simulink model "mu_nonlinear_sim"  (R2026b)
settings: Solver=VariableStepAuto
InitFcn:
  | seaDir=fileparts(get_param(bdroot,'FileName'));if isfile(fullfile(seaDir,'..','collaudo_simulink.m')),addpath(fullfile(seaDir,'..'));else,addpath(fullfile(seaDir,'..','..','File_di_Funzioni_Progetto-Accorpati'));end;collaudo_simulink(bdroot);
model workspace (MAT data in the model file):
  A = [0  0  1  0  0  0  0  0  0  0  0  0  0  0; 0  0  0  1  0  0  0  0  0  0  0  0  0  0; -287.975  563.713333333  0  0  312.5  -583.333333333  0  0  0  0  0  0  0  0; 704.641666667  -1838.18666667  0  0  -729.166666667  1916.66666667  0  0  0  0  0  0  0  0; 0  0  0  0  0  0  1  0  0  0  0  0  0  0; 0  0  0  0  0  0  0  1  0  0  0  0  0  0; 5000  0  0  0  -5000  0  -2  0  0  -156.25  651.041666667  0  0  0; 0  4000  0  0  0  -4000  0  -2  0  0  0  0  -156.25  651.041666667; 0  0  0  0  0  0  0  0  -197.333333333  -79.1666666667  -52.0833333333  0  0  0; 0  0  0  0  0  0  0  0  128  0  0  0  0  0; 0  0  0  0  0  0  0  0  0  32  0  0  0  0; 0  0  0  0  0  0  0  0  0  0  0  -197.333333333  -79.1666666667  -52.0833333333; 0  0  0  0  0  0  0  0  0  0  0  128  0  0; 0  0  0  0  0  0  0  0  0  0  0  0  32  0]
  Ak1 = [-59053.7551233 -15060.4417981 -247384.802166 -33683.9989112 -58744.8100055 -15054.8155194 -240737.427005 -34798.0678804 -380.093427931 -2.64528507321e-11 -2.86785014033e-11 -70.1772916652 ... (324 elements, 18x18)]
  Ak2 = [-66482.5138518 58859.9072435 -3939180219.02 8861329774.8 0.00962184169638 0.0021126060022 -0.307210144554 -0.149393411391 -808382.886676 -1.97154781154e-06 -5.5678995061e-07 -402416.605778 ... (484 elements, 22x22)]
  Aplant = [0  0  1  0  0  0  0  0  0  0  0  0  0  0; 0  0  0  1  0  0  0  0  0  0  0  0  0  0; -287.975  563.713333333  0  0  312.5  -583.333333333  0  0  0  0  0  0  0  0; 704.641666667  -1838.18666667  0  0  -729.166666667  1916.66666667  0  0  0  0  0  0  0  0; 0  0  0  0  0  0  1  0  0  0  0  0  0  0; 0  0  0  0  0  0  0  1  0  0  0  0  0  0; 5000  0  0  0  -5000  0  -2  0  0  -156.25  651.041666667  0  0  0; 0  4000  0  0  0  -4000  0  -2  0  0  0  0  -156.25  651.041666667; 0  0  0  0  0  0  0  0  -197.333333333  -79.1666666667  -52.0833333333  0  0  0; 0  0  0  0  0  0  0  0  128  0  0  0  0  0; 0  0  0  0  0  0  0  0  0  32  0  0  0  0; 0  0  0  0  0  0  0  0  0  0  0  -197.333333333  -79.1666666667  -52.0833333333; 0  0  0  0  0  0  0  0  0  0  0  128  0  0; 0  0  0  0  0  0  0  0  0  0  0  0  32  0]
  B = [0  0; 0  0; 0  0; 0  0; 0  0; 0  0; 0  0; 0  0; 8  0; 0  0; 0  0; 0  8; 0  0; 0  0]
  Bk1 = [-41971.7925923  -11081.1547486; -10702.5482864  -2862.34383586; -175622.627059  -46334.0254179; -24431.1418067  -6701.2370812; -41752.2098485  -11023.2672925; -10698.572028  -2860.7387349; -174656.417143  -46079.7084794; -24722.2969121  -6774.18550393; 2.40651657511e-11  6.37680376741e-12; -1.88006601576e-11  -4.97364228434e-12; -2.03813396558e-11  -5.41993380938e-12; 1.08535358931e-11  2.8764122053e-12; 9.45959622107e-14  1.502238924e-14; 6.09740887216e-12  1.59629499127e-12; 1  4.38779674844e-13; -1.60225617681e-11  0.999999999996; 2.09437869826e-11  5.51387120759e-12; 7.22259613326e-12  1.92024020066e-12]
  Bk2 = [-1.469715923e-05  -5.03392161697e-06  66481.5344792  -58860.9820595; -1.60967680897e-05  -5.61949285195e-06  -58860.9820595  240347.325722; 0.0248933110796  0.0149679212434  3939075365.52  -9206373341.64; -2.94053204371  -1.03244143942  -8861110672.09  30611501156.9; 8.38580299227e-11  2.88681171192e-11  -0.00961625066757  -0.0107019560654; 1.81369365811e-11  6.22825118722e-12  -0.00211139708193  -0.00220551516129; -2.44265911788e-09  -8.38310293341e-10  5000.30704734  0.311108840593; -1.28586131714e-09  -4.47766304456e-10  0.149307574964  4000.17933035; -3.3652681538e-15  -7.79427381522e-16  1.22929631189e-07  5.43969913477e-07; -1.54732535343e-14  -5.27443674215e-15  1.97051724139e-06  1.69233324755e-06; -5.91421615725e-15  -1.60957708692e-15  5.56404379394e-07  6.44318326468e-07; 6.60057972656e-15  2.06268116455e-15  -1.4300097113e-07  -1.54855124633e-06; -2.97654953502e-15  2.4134857998e-16  -3.49285009668e-07  4.31276255736e-07; -2.94350008791e-14  -1.06328803069e-14  3.2069323084e-06  4.47049231709e-06; 2  -2.928912043e-15  9.46335392933e-07  1.16503477027e-06; 2.28965391755e-14  7.37138472727e-15  -2.63923776257e-06  -2.83353275499e-06; 4.99201069125e-16  2  -6.74353253191e-08  -1.3033050226e-07; 2.3272465043e-15  7.76116322822e-16  -2.74324508576e-07  -3.61337801409e-07; -1.06347642829e-12  -3.65803490785e-13  1.00012374907  0.000134433844037; -3.40933375091e-13  -1.18005737123e-13  3.9069788798e-05  1.00004517384; 3.33367848603e-15  1.22297283889e-15  -4.2121398571e-07  -3.40032598636e-07; 2.80802881661e-16  3.33510230464e-16  -8.09517197876e-08  -4.97664970119e-08]
  Bplant = [0  0  0  0  0  0  0  0; 0  0  0  0  0  0  0  0; 0  0  6.25  -14.5833333333  6.25  -14.5833333333  0  0; 0  0  -14.5833333333  47.9166666667  -14.5833333333  47.9166666667  0  0; 0  0  0  0  0  0  0  0; 0  0  0  0  0  0  0  0; 0  0  0  0  0  0  0  0; 0  0  0  0  0  0  0  0; 8  0  0  0  0  0  8  0; 0  0  0  0  0  0  0  0; 0  0  0  0  0  0  0  0; 0  8  0  0  0  0  0  8; 0  0  0  0  0  0  0  0; 0  0  0  0  0  0  0  0]
  C = [1  0  0  0  0  0  0  0  0  0  0  0  0  0; 0  1  0  0  0  0  0  0  0  0  0  0  0  0; 0  0  0  0  1  0  0  0  0  0  0  0  0  0; 0  0  0  0  0  1  0  0  0  0  0  0  0  0]
  Ck1 = [-47.5116784914  -5.78209213287  -5.13823657239  -1.08700411022  -2.20352010323  2.66425180559  -0.125034922339  0.185992241592  -0.927741743434  -1.56246668763  -3.63799575165  0.692641920355  1.31947037114  4.18733038989  131.03488926  -0.481581356595  185.834513399  7.27974776868; -8.77216145816  -28.2907119683  -1.33504865248  -1.92106436843  2.82254774196  -9.29393606241  0.15386065621  -0.640740236363  0.661174214458  1.22612259058  3.63119486569  -2.61713226851  -4.77953727904  -14.316530373  8.32978038536  120.88787202  7.40561859226  167.361916298]
  Ck2 = [-101047.860834  -35271.4725267  -10213.2861669  -3422.70914383  -726.305194157  -2764.75614997  -134.44732536  -147.179762398  -1026.38324203  -1695.61454007  -3888.56222989  -577.341883828  -1018.80852496  -3004.81089551  37664.9906718  104577.837385  12946.0064238  38967.5403937  -276393.79928  -109642.430073  -16958.192986  -8226.89474918; -50302.0757223  -17755.3765506  -5087.46688004  -1714.88123493  -339.218722956  -1461.38985543  -65.6273114827  -77.9347122137  -507.469938959  -837.275262695  -1911.06705358  -299.403482778  -530.388353735  -1580.54605831  18756.946896  52040.0304562  6501.42413314  19681.1036111  -137452.475336  -55605.1885505  -8506.38250139  -4027.49208907]
  Cplant = [1  0  0  0  0  0  0  0  0  0  0  0  0  0; 0  1  0  0  0  0  0  0  0  0  0  0  0  0; 0  0  0  0  1  0  0  0  0  0  0  0  0  0; 0  0  0  0  0  1  0  0  0  0  0  0  0  0]
  D = [0  0; 0  0; 0  0; 0  0]
  Dk1 = [0  0; 0  0]
  Dk2 = [0  0  0  0; 0  0  0  0]
  Dplant = [0  0  0  0  0  0  0  0; 0  0  0  0  0  0  0  0; 0  0  0  0  0  0  0  0; 0  0  0  0  0  0  0  0]
  Gact = ss
  Gact.IOSize_ = [1 1]
  Gact.Data_ = ltipack.ssdata
  Gact.Data_.a = [-197.333333333  -79.1666666667  -52.0833333333  0  0  0; 128  0  0  0  0  0; 0  32  0  0  0  0; 0  0  0  -197.333333333  -79.1666666667  -52.0833333333; 0  0  0  128  0  0; 0  0  0  0  32  0]
  Gact.Data_.c = [0 -1.5625 6.51041666667 0 0 0]
  Gact.Data_.dx0 = [0; 0; 0; 0; 0; 0]
  Gact.Data_.x0 = [0; 0; 0; 0; 0; 0]
  Gact.Data_.b = [8; 0; 0; 0; 0; 0]
  Gact.Data_.d = 0
  Gact.Data_.u0 = 0
  Gact.Data_.y0 = 0
  Gact.Data_.Delay.Input = 0
  Gact.Data_.Delay.Output = 0
  Gact.Data_.Delay.Internal = []
  Gact.Data_.Ts = 0
  Gact1 = ss
  Gact1.IOSize_ = [1 1]
  Gact1.Data_ = ltipack.ssdata
  Gact1.Data_.a = [-197.333333333  -79.1666666667  -52.0833333333  0  0  0; 128  0  0  0  0  0; 0  32  0  0  0  0; 0  0  0  -197.333333333  -79.1666666667  -52.0833333333; 0  0  0  128  0  0; 0  0  0  0  32  0]
  Gact1.Data_.c = [0 -1.5625 6.51041666667 0 0 0]
  Gact1.Data_.dx0 = [0; 0; 0; 0; 0; 0]
  Gact1.Data_.x0 = [0; 0; 0; 0; 0; 0]
  Gact1.Data_.b = [8; 0; 0; 0; 0; 0]
  Gact1.Data_.d = 0
  Gact1.Data_.u0 = 0
  Gact1.Data_.y0 = 0
  Gact1.Data_.Delay.Input = 0
  Gact1.Data_.Delay.Output = 0
  Gact1.Data_.Delay.Internal = []
  Gact1.Data_.Ts = 0
  Gact2 = ss
  Gact2.IOSize_ = [1 1]
  Gact2.Data_ = ltipack.ssdata
  Gact2.Data_.a = [-197.333333333  -79.1666666667  -52.0833333333  0  0  0; 128  0  0  0  0  0; 0  32  0  0  0  0; 0  0  0  -197.333333333  -79.1666666667  -52.0833333333; 0  0  0  128  0  0; 0  0  0  0  32  0]
  Gact2.Data_.c = [0 0 0 0 -1.5625 6.51041666667]
  Gact2.Data_.dx0 = [0; 0; 0; 0; 0; 0]
  Gact2.Data_.x0 = [0; 0; 0; 0; 0; 0]
  Gact2.Data_.b = [0; 0; 0; 8; 0; 0]
  Gact2.Data_.d = 0
  Gact2.Data_.u0 = 0
  Gact2.Data_.y0 = 0
  Gact2.Data_.Delay.Input = 0
  Gact2.Data_.Delay.Output = 0
  Gact2.Data_.Delay.Internal = []
  Gact2.Data_.Ts = 0
  K = [254.334027129  15.8581705289  18.8630740974  3.80874559615  -166.282584787  -12.9480516363  -1.29863159415  -0.917623908585  11.5550875651  22.0162263478  42.3100515756  -0.973759695773  -2.3551817304  -13.4833901328; 14.9301350665  213.753684859  4.69692491423  7.32991673361  -5.53696181317  -143.459502962  -0.645259935367  1.32092931509  -0.973759695773  -2.22266457033  -10.9075066091  14.3308977175  28.5410559812  79.9065315403]
  Ki = [-44.6778372022  1.97252704227; -1.97252704227  -44.6778372022]
  Kmu = ss
  Kmu.IOSize_ = [2 4]
  Kmu.Data_ = ltipack.ssdata
  Kmu.Data_.a = [-0.665232802392 -1.47380282002 -1.22221847669e-15 -4.48274447352e-16 3.2327584929e-05 -0.0206808301531 -0.00529526796856 -0.517967014923 -13.8634978319 26.8745194974 0.0193720277147 0.64558333357 ... (58564 elements, 242x242)]
  Kmu.Data_.c = [3.3783170995 -5.8072266427 2.84420711761 -4.48632603242 -1.18767506872 -1.0721534743 -0.902312590905 -2.93021975862 -2.7744790437 5.00986645551 -2.58581192448 4.60146909465 ... (484 elements, 2x242)]
  Kmu.Data_.dx0 = [0; 0; 0; 0; 0; 0; 0; 0; 0; 0; 0; 0; 0; 0; 0; 0; 0; 0; 0; 0; 0; 0; 0; 0; 0; 0; 0; 0; 0; 0; 0; 0; 0; 0; 0; 0; 0; 0; 0; 0; 0; 0; 0; 0; 0; 0; 0; 0; 0; 0; 0; 0; 0; 0; 0; 0; 0; 0; 0; 0; 0; 0; 0; 0; 0; 0; 0; 0; 0; 0; 0; 0; 0; 0; 0; 0; 0; 0; 0; 0; 0; 0; 0; 0; 0; 0; 0; 0; 0; 0; 0; 0; 0; 0; 0; 0; 0; 0; 0; 0; 0; 0; 0; 0; 0; 0; 0; 0; 0; 0; 0; 0; 0; 0; 0; 0; 0; 0; 0; 0; 0; 0; 0; 0; 0; 0; 0; 0; 0; 0; 0; 0; 0; 0; 0; 0; 0; 0; 0; 0; 0; 0; 0; 0; 0; 0; 0; 0; 0; 0; 0; 0; 0; 0; 0; 0; 0; 0; 0; 0; 0; 0; 0; 0; 0; 0; 0; 0; 0; 0; 0; 0; 0; 0; 0; 0; 0; 0; 0; 0; 0; 0; 0; 0; 0; 0; 0; 0; 0; 0; 0; 0; 0; 0; 0; 0; 0; 0; 0; 0; 0; 0; 0; 0; 0; 0; 0; 0; 0; 0; 0; 0; 0; 0; 0; 0; 0; 0; 0; 0; 0; 0; 0; 0; 0; 0; 0; 0; 0; 0; 0; 0; 0; 0; 0; 0; 0; 0; 0; 0; 0; 0]
  Kmu.Data_.x0 = [0; 0; 0; 0; 0; 0; 0; 0; 0; 0; 0; 0; 0; 0; 0; 0; 0; 0; 0; 0; 0; 0; 0; 0; 0; 0; 0; 0; 0; 0; 0; 0; 0; 0; 0; 0; 0; 0; 0; 0; 0; 0; 0; 0; 0; 0; 0; 0; 0; 0; 0; 0; 0; 0; 0; 0; 0; 0; 0; 0; 0; 0; 0; 0; 0; 0; 0; 0; 0; 0; 0; 0; 0; 0; 0; 0; 0; 0; 0; 0; 0; 0; 0; 0; 0; 0; 0; 0; 0; 0; 0; 0; 0; 0; 0; 0; 0; 0; 0; 0; 0; 0; 0; 0; 0; 0; 0; 0; 0; 0; 0; 0; 0; 0; 0; 0; 0; 0; 0; 0; 0; 0; 0; 0; 0; 0; 0; 0; 0; 0; 0; 0; 0; 0; 0; 0; 0; 0; 0; 0; 0; 0; 0; 0; 0; 0; 0; 0; 0; 0; 0; 0; 0; 0; 0; 0; 0; 0; 0; 0; 0; 0; 0; 0; 0; 0; 0; 0; 0; 0; 0; 0; 0; 0; 0; 0; 0; 0; 0; 0; 0; 0; 0; 0; 0; 0; 0; 0; 0; 0; 0; 0; 0; 0; 0; 0; 0; 0; 0; 0; 0; 0; 0; 0; 0; 0; 0; 0; 0; 0; 0; 0; 0; 0; 0; 0; 0; 0; 0; 0; 0; 0; 0; 0; 0; 0; 0; 0; 0; 0; 0; 0; 0; 0; 0; 0; 0; 0; 0; 0; 0; 0]
  Kmu.Data_.b = [0.00348017534504 0.0155187296828 -1.12970714394e-12 -4.00980133056e-13 -0.00296740301472 -0.0167004632251 0.00283691752204 0.001803502039 0.00204485285148 -0.000516488693839 0.513240971973 0.0925801218799 ... (968 elements, 242x4)]
  Kmu.Data_.d = [0  0  0  0; 0  0  0  0]
  Kmu.Data_.u0 = [0; 0; 0; 0]
  Kmu.Data_.y0 = [0; 0]
  Kmu.Data_.Delay.Input = [0; 0; 0; 0]
  Kmu.Data_.Delay.Output = [0; 0]
  Kmu.Data_.Delay.Internal = []
  Kmu.Data_.Ts = 0
  Kpid = ss
  Kpid.IOSize_ = [2 4]
  Kpid.Data_ = ltipack.ssdata
  Kpid.Data_.a = [0  0  0  0; 0  -57593.2995109  0  0; 0  0  0  0; 0  0  0  -0.329919928085]
  Kpid.Data_.c = [6.4783768333  247678.711236  0  0; 0  0  6.03188457292  -0.555209004946]
  Kpid.Data_.dx0 = [0; 0; 0; 0]
  Kpid.Data_.x0 = [0; 0; 0; 0]
  Kpid.Data_.b = [1  0  -1  0; -10.2124088214  0  57593.2995109  0; 0  1  0  -1; 0  -0.370103018763  0  0.329919928085]
  Kpid.Data_.d = [46.09798011  0  -247695.83824  0; 0  -0.622584779977  0  -6.02512572971]
  Kpid.Data_.u0 = [0; 0; 0; 0]
  Kpid.Data_.y0 = [0; 0]
  Kpid.Data_.Delay.Input = [0; 0; 0; 0]
  Kpid.Data_.Delay.Output = [0; 0]
  Kpid.Data_.Delay.Internal = []
  Kpid.Data_.Ts = 0
  Kx = [269.29854219  18.7569204553  20.3465743072  4.21621347174  -167.135644221  -13.7370160239  -1.23948523054  -0.937049335048  11.6520090072  22.2361236584  43.3764212876  -0.976831004507  -2.36858741141  -13.665069792; 18.5296585008  219.858519907  5.19353276352  7.65247929484  -6.07863263477  -142.076957605  -0.661137562181  1.43283057057  -0.976831004508  -2.23596989408  -11.0675872205  14.4349878373  28.7952856037  81.4581543362]
  L = [22.7086027083  -21.7936009117  9.04408034457  -5.52266339377; -21.7936009117  85.6043203583  -6.92262592935  23.4709799065; 551.468438951  -1274.37297548  233.268454557  -349.376578167; -1278.38675006  4200.93517611  -381.596753676  1210.55343734; 9.04408034457  -6.92262592934  64.3796319985  -3.42186433889; -5.52266339377  23.4709799065  -3.42186433889  79.1961089718; 724.131288886  -934.103630678  2143.08215542  -313.448848015; -755.873627778  2801.52113681  -390.276085477  3432.55977028; -0.415262976271  -2.25405487396  -35.1145525411  -1.7286492798; 24.3199274492  14.4090239346  -92.1365142338  -0.288628866805; -30.0664339157  -12.6731701589  207.827992725  4.7947871058; -1.9578954483  4.81325829224  -1.70248790351  -30.0318182029; 11.5399257048  -9.16509666779  1.36047325197  -101.985096573; -9.75889255449  -0.59061749336  2.61696327045  207.422378213]
  Nr = [54.3883750199  -1.27699836083; 3.40681303355  51.6920123589]
  m2_eff = 0.8
  taubar = [5.76661684783e-16; 1.44165421196e-16]
  x0plant = [0; 0; 0; 0; 0; 0; 0; 0; 0; 0; 0; 0; 0; 0]
  xbar = [1.57079632679; 0; 0; 0; 1.57079632679; 3.60413552989e-18; 0; 0]
libraries: cstblocks_lti x3
settings Model: Creator=rebec  LastModifiedBy=aless

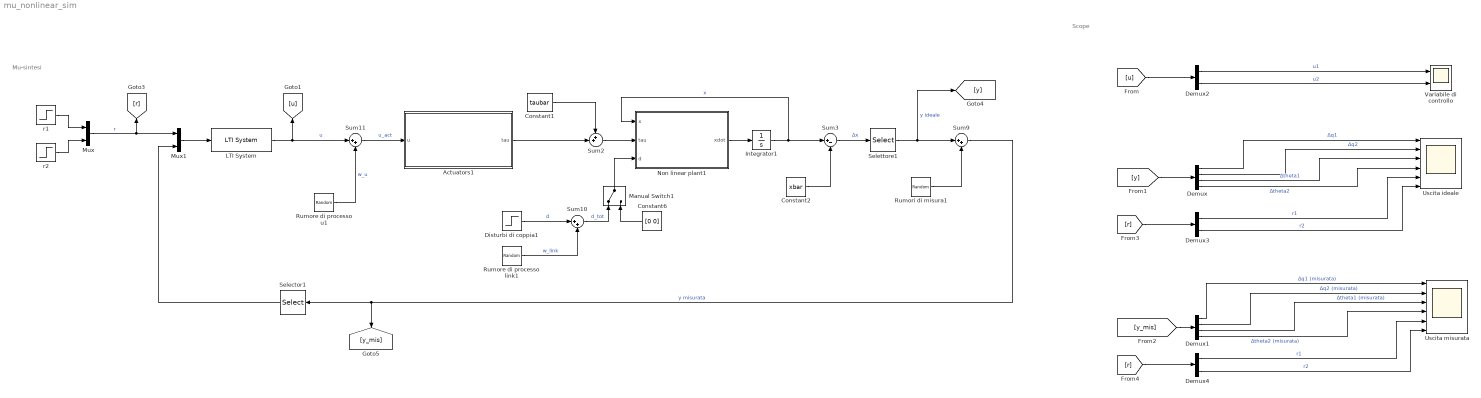
== system mu_nonlinear_sim ==
  note: Scope
  note: Mu-sintesi
  Actuators1 : Subsystem
  Constant1 : Constant  Value=taubar
  Constant2 : Constant  Value=xbar
  Constant6 : Constant  Value=[0 0]
  Demux : Demux
  Demux1 : Demux
  Demux2 : Demux  Outputs=2
  Demux3 : Demux  Outputs=2
  Demux4 : Demux  Outputs=2
  Disturbi di coppia1 : Step  Time=[1 1]  InitialValue=[0 0]  FinalValue=[0.5 0]  SampleTime=0
  Integrator1 : Integrator  InitialCondition=xbar
  LTI System : cstblocks_lti/LTI System  sys=Kmu  IC=[]  PadeOrder=0
      settings: LibrarySourceBlock=cstblocks/LTI System
  Manual Switch1 : ManualSwitch
  Mux : Mux  Inputs=2
  Mux1 : Mux  Inputs=2
  Non linear plant1 : Subsystem
  Rumore di processo link1 : RandomNumber  Mean=[0 0]  Variance=[0.01 0.01]  Seed=20260826  SampleTime=0.002
  Rumore di processo u1 : RandomNumber  Mean=[0 0]  Variance=[0.01 0.01]  Seed=20260826  SampleTime=0.002
  Rumori di misura1 : RandomNumber  Mean=[0 0 0 0]  Variance=[(0.05*pi/180)^2 (0.05*pi/180)^2 (0.05*pi/180)^2 (0.05*pi/180)^2]  Seed=20260826  SampleTime=0.002
  Selector1 : Selector  InputPortWidth=4  IndexOptions=Index vector (dialog)  Indices=[1 2]  OutputSizes=1  RuntimeRangeChecks=off
  Selettore1 : Selector  InputPortWidth=8  IndexOptions=Index vector (dialog)  Indices=[1 2 5 6]  OutputSizes=1  RuntimeRangeChecks=off
  Sum10 : Sum  Inputs=|++
  Sum11 : Sum  Inputs=|++
  Sum2 : Sum  Inputs=++|
  Sum3 : Sum  Inputs=|+-
  Sum9 : Sum  Inputs=|++
  Uscita ideale : Scope  NumInputPorts=6
      settings: Title=Uscita ideale (mu NL)  ActiveDisplayYMinimum=-0.088271118920575181  ActiveDisplayYMaximum=0.23303114019935003  YLabel=y (rad)
  Uscita misurata : Scope  NumInputPorts=6
      settings: Title=Uscita misurata (mu NL)  ActiveDisplayYMinimum=-0.11442029066688837  ActiveDisplayYMaximum=0.16914890182413583  YLabel=y (rad)
  Variabile di controllo : Scope  NumInputPorts=2
      settings: Title=Variabili di controllo (mu NL)  ActiveDisplayYMinimum=-14.512240124873713  ActiveDisplayYMaximum=7.6680416810083489  YLabel=u (Nm)  DataLoggingVariableName=ScopeData2
  r1 : Step  FinalValue=5*pi/180  SampleTime=0
  r2 : Step  FinalValue=0  SampleTime=0
  wires:
  Manual Switch1/1 -> Non linear plant1/3(d)
  Selector1/1 -> Mux1/2
  r2/1 -> Mux/2
  Sum9/1 -> [y_mis], Selector1/1  "y misurata"
  r1/1 -> Mux/1
  Integrator1/1 -> Non linear plant1/1(x), Sum3/1  "x"
  Constant2/1 -> Sum3/2
  Sum3/1 -> Selettore1/1  "Δx"
  Sum10/1 -> Manual Switch1/1  "d_tot"
  Constant1/1 -> Sum2/1
  Sum2/1 -> Non linear plant1/2(tau)
  Constant6/1 -> Manual Switch1/2
  Sum11/1 -> Actuators1/1(u)  "u_act"
  Mux/1 -> Mux1/1, [r]  "r"
  Actuators1/1(tau) -> Sum2/2
  Rumore di processo u1/1 -> Sum11/2  "w_u"
  LTI System/1 -> Sum11/1, [u]  "u"
  Selettore1/1 -> Sum9/1, [y]  "y ideale"
  Rumore di processo link1/1 -> Sum10/2  "w_link"
  Disturbi di coppia1/1 -> Sum10/1  "d"
  Mux1/1 -> LTI System/1
  Non linear plant1/1(xdot) -> Integrator1/1
  [y_mis] -> Demux1/1
  Demux4/2 -> Uscita misurata/6  "r2"
  Demux1/4 -> Uscita misurata/4  "Δtheta2 (misurata)"
  [r] -> Demux3/1
  Demux1/2 -> Uscita misurata/2  "Δq2 (misurata)"
  Demux4/1 -> Uscita misurata/5  "r1"
  [r] -> Demux4/1
  Demux/3 -> Uscita ideale/3  "Δtheta1"
  Demux/4 -> Uscita ideale/4  "Δtheta2"
  [y] -> Demux/1
  Demux/1 -> Uscita ideale/1  "Δq1"
  Demux/2 -> Uscita ideale/2  "Δq2"
  Demux2/1 -> Variabile di controllo/1  "u1"
  Demux3/2 -> Uscita ideale/6  "r2"
  Demux1/3 -> Uscita misurata/3  "Δtheta1 (misurata)"
  Demux3/1 -> Uscita ideale/5  "r1"
  Demux2/2 -> Variabile di controllo/2  "u2"
  [u] -> Demux2/1
  Demux1/1 -> Uscita misurata/1  "Δq1 (misurata)"
  Rumori di misura1/1 -> Sum9/2

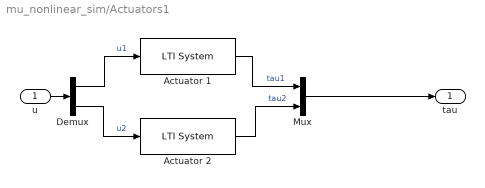
== system mu_nonlinear_sim/Actuators1 ==
  u : Inport
  Actuator 1 : cstblocks_lti/LTI System  sys=Gact1  IC=[]  PadeOrder=0
      settings: LibrarySourceBlock=cstblocks/LTI System
  Actuator 2 : cstblocks_lti/LTI System  sys=Gact2  IC=[]  PadeOrder=0
      settings: LibrarySourceBlock=cstblocks/LTI System
  Demux : Demux  Outputs=2
  Mux : Mux  Inputs=2
  tau : Outport
  wires:
  Actuator 2/1 -> Mux/2  "tau2"
  Demux/2 -> Actuator 2/1  "u2"
  u/1 -> Demux/1
  Demux/1 -> Actuator 1/1  "u1"
  Mux/1 -> tau/1
  Actuator 1/1 -> Mux/1  "tau1"

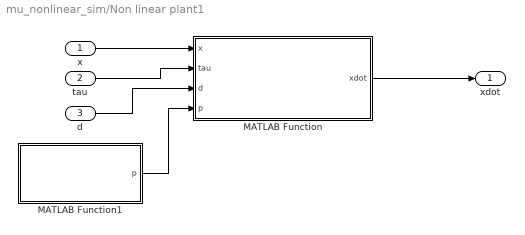
== system mu_nonlinear_sim/Non linear plant1 ==
  x : Inport
  tau : Inport  Port=2
  d : Inport  Port=3
  MATLAB Function : MATLAB Function  TreatAsAtomicUnit=on
  MATLAB Function1 : MATLAB Function  TreatAsAtomicUnit=on
  xdot : Outport
  wires:
  x/1 -> MATLAB Function/1(x)
  tau/1 -> MATLAB Function/2(tau)
  MATLAB Function/1(xdot) -> xdot/1
  MATLAB Function1/1(p) -> MATLAB Function/4(p)
  d/1 -> MATLAB Function/3(d)

== matlab function mu_nonlinear_sim/Non linear plant1/MATLAB Function ==
  data: x input; xdot output; tau input; d input; p input
function xdot = sea_nonlinear_rhs_with_link_disturbance(x, tau, d, p)
%SEA_NONLINEAR_RHS_WITH_LINK_DISTURBANCE SEA dynamics with link torque D.
%   TAU remains the motor-side input; D is an external link-side joint
%   torque entering with positive sign in the link equation.

assert(numel(x) == 8, ...
    'sea_nonlinear_rhs_with_link_disturbance:InvalidState', ...
    'The state must contain exactly eight elements.');
assert(numel(tau) == 2 && numel(d) == 2, ...
    'sea_nonlinear_rhs_with_link_disturbance:InvalidInput', ...
    'Both tau and d must contain exactly two elements.');
x = reshape(x, 8, 1);
tau = reshape(tau, 2, 1);
d = reshape(d, 2, 1);

q = x(1:2);
qdot = x(3:4);
theta = x(5:6);
thetadot = x(7:8);
M = sea_link_inertia(q, p);
C = sea_coriolis(q, qdot, p);
G = sea_gravity(q, p);
tauElastic = sea_elastic_torque(q, theta, p);

qddot = M \ (tauElastic + d - C * qdot - G);
thetaddot = p.Jm \ (tau - p.Bm * thetadot - tauElastic);
xdot = [qdot; qddot; thetadot; thetaddot];
end

== matlab function mu_nonlinear_sim/Non linear plant1/MATLAB Function1 ==
  data: p output Bus: slBus1; m2_eff parameter
function p = sea_params_nominal(m2_eff)
%SEA_PARAMS_NOMINAL Nominal mechanical parameters of the 2R SEA robot.
%   P = SEA_PARAMS_NOMINAL returns the values stated by the official
%   assignment. Matrices follow the joint order [joint 1; joint 2].

p.m1 = 1.0;                   % kg
p.m2 = m2_eff;                   % kg
p.l1 = 0.4;                   % m
p.l2 = 0.3;                   % m
p.Jm = diag([0.01, 0.01]);    % kg*m^2
p.Bm = diag([0.02, 0.02]);    % N*m*s/rad
p.Ks = diag([50, 40]);        % N*m/rad
p.g = 9.81;                   % m/s^2
end
